simulink library "MFMbody_roadSurface"  (R2025a)
settings: Solver=VariableStepAuto  StartTime=0.0  StopTime=10.0  RelTol=1e-3
undefined symbols (not defined in the file): fcontactpatch, LorR, road_file, Scene, SceneData, Vehicle, X, Y, Z
libraries: sm_lib x21, nesl_utility x12, $bdroot x7
Description:
  | Component of Simscape Vehicle Templates Library
  | 
  | Copyright 2018-2026 The MathWorks, Inc.
settings Model: Creator=smiller  LastModifiedBy=smiller
settings OptimizationCC: ReuseModelBlockBuffer=off
settings ModelReferenceCC: EnableRefExpFcnMdlSchedulingChecks=on
settings RTWCC: GPUComputeCapability=3.5

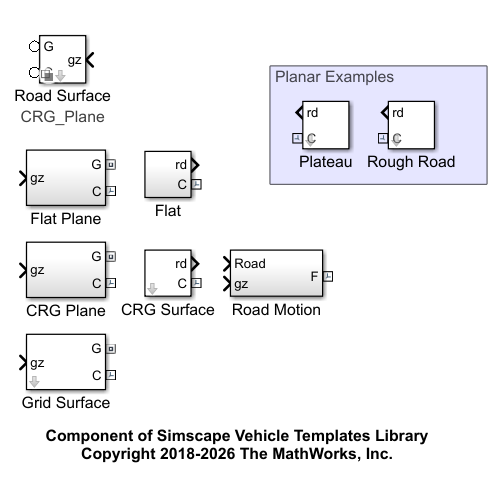
[thumbnail: Simulink's stored preview of the top-level diagram]
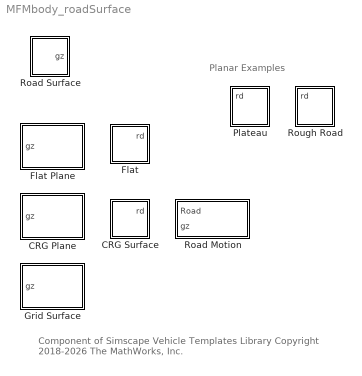
== system MFMbody_roadSurface ==
  note: Planar Examples
  note: Component of Simscape Vehicle Templates Library
      | Copyright 2018-2026 The MathWorks, Inc.
  CRG Plane : Subsystem
  CRG Surface : Subsystem  mask{road_file=road_file, LRind=LorR}
      mask prompts: road_file "Road File Name"; LRind "Index for Left (1) or Right (2)"
      mask init:
      | set_param([gcb '/Contact Plane'],'crg_file',road_file);
  Flat : Subsystem
  Flat Plane : Subsystem
  Grid Surface : Subsystem  mask{grid_file=Vehicle.Chassis.TireA1.roadFile.Value}
      mask prompts: grid_file "Road File Name (stl)"
      mask init:
      | parStr = ['Scene.' strrep(grid_file,'.stl','.gsd')];
      | 
      | set_param([gcb '/Grid Surface'],...
      |     'XGridVector',[parStr '.xg'],...
      |     'YGridVector',[parStr '.yg'],...
      |     'ZHeights',[parStr '.z_heights']);
  Plateau : Subsystem  mask{LRind=LorR}
      mask prompts: LRind "Index for Left (1) or Right (2)"
  Road Motion : Subsystem
  Road Surface : Subsystem  Variant=on  VariantControlMode=label  VariantControl=Choice  LabelModeActiveChoice=CRG_Plane  mask{popup_leftRight=Left}
      mask prompts: popup_leftRight "Left/Right"
      mask init:
      | LorR = 1;
      | if(strcmpi(get_param(gcb,'popup_leftRight'),'right'))
      |     LorR = 2;
      | end
      settings: AttributesFormatString=%<LabelModeActiveChoice>
      mask TypeOptions popup_leftRight: Left | Right
      mask Display: disp(' ')
  Rough Road : Subsystem  mask{LRind=LorR}
      mask prompts: LRind "Index for Left (1) or Right (2)"

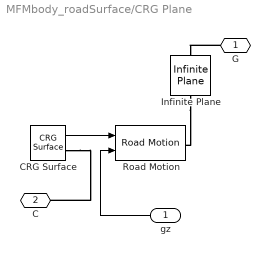
== system MFMbody_roadSurface/CRG Plane ==
  gz : Inport
  CRG Surface : $bdroot/CRG Surface  VariantControl=CRG_Surface  road_file=road_file  LRind=LorR
  Infinite Plane : sm_lib/Curves and Surfaces/Infinite Plane  GraphicType=Rectangle  GraphicPlaneWidth=1  GraphicPlaneWidthUnits=m  GraphicPlaneHeight=1  GraphicPlaneHeightUnits=m  GraphicVisPropType=SimpleVisualProperties  GraphicDiffuseColor=Visual.TireContactPlane.clr  GraphicOpacity=Visual.TireContactPlane.opc  GraphicSpecularColor=[0.5 0.5 0.5 1.0]  GraphicAmbientColor=[0.15 0.15 0.15 1.0]  GraphicEmissiveColor=[0.0 0.0 0.0 1.0]  GraphicShininess=75
  Road Motion : $bdroot/Road Motion  SystemSampleTime=-1  VariantActivationTime=update diagram  EmptyChoice=off  PassThrough=off  PassThroughVariantControl=(default)  EmptyChoiceVariantControl=(default)  AllowFlexibleInterface=on  Latency=0  AutoFrameSizeCalculation=off
  G : PMIOPort  Side=Right
  C : PMIOPort  Port=2  Side=Right
  wires:
  gz/1 -> Road Motion/2
  CRG Surface/1 -> Road Motion/1
  connections:
  CRG Surface/RConn1 -- C/RConn1
  Infinite Plane/LConn1 -- Road Motion/RConn1
  G/RConn1 -- Infinite Plane/RConn1

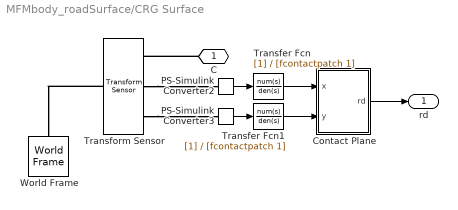
== system MFMbody_roadSurface/CRG Surface ==
  Contact Plane : Subsystem  mask{crg_file=road_file}
      mask prompts: crg_file "CRG Road File"
      mask init:
      | crg = crg_read(crg_file);
      | crg = rmfield(crg,'ct');
      | crg = rmfield(crg,'struct');
  PS-Simulink Converter2 : nesl_utility/PS-Simulink Converter  PhysicalDomain=network_engine_domain  SubClassName=ps_output  LeftPortType=input  RightPortType=output  PseudoPeriodic=off  Frequencies=[]  VectorFormat=inherit  Unit=inherit  AffineConversion=off
  PS-Simulink Converter3 : nesl_utility/PS-Simulink Converter  PhysicalDomain=network_engine_domain  SubClassName=ps_output  LeftPortType=input  RightPortType=output  PseudoPeriodic=off  Frequencies=[]  VectorFormat=inherit  Unit=inherit  AffineConversion=off
  Transfer Fcn : TransferFcn  Denominator=[fcontactpatch 1]
  Transfer Fcn1 : TransferFcn  Denominator=[fcontactpatch 1]
  Transform Sensor : sm_lib/Frames and Transforms/Transform Sensor  MeasurementFrame=World  RotationSequence=XYX  SenseAngle=off  SenseAxis=off  SenseQ=off  SenseR=off  SenseRotationSequence=off  SenseOmegaX=off  SenseOmegaY=off  SenseOmegaZ=off  SenseOmega=off  SenseQDot=off  SenseRDot=off  SenseRotationSequenceDot=off  SenseAlphaX=off  SenseAlphaY=off  SenseAlphaZ=off  SenseAlpha=off  SenseQDDot=off  SenseRDDot=off  SenseX=on  SenseY=on  SenseZ=off  SenseXYZ=off  SenseRad=off  SenseAzim=off  SenseDist=off  SenseInc=off  SenseXDot=off  SenseYDot=off  SenseZDot=off  SenseXYZDot=off  SenseRadDot=off  SenseAzimDot=off  SenseDistDot=off  SenseIncDot=off  SenseXDDot=off  SenseYDDot=off  SenseZDDot=off  SenseXYZDDot=off  SenseRadDDot=off  SenseAzimDDot=off  SenseDistDDot=off  SenseIncDDot=off
  World Frame : sm_lib/Frames and Transforms/World Frame
  C : PMIOPort  Side=Right
  rd : Outport
  wires:
  PS-Simulink Converter2/1 -> Transfer Fcn/1
  PS-Simulink Converter3/1 -> Transfer Fcn1/1
  Transfer Fcn/1 -> Contact Plane/1(x)
  Transfer Fcn1/1 -> Contact Plane/2(y)
  Contact Plane/1(rd) -> rd/1
  connections:
  Transform Sensor/LConn1 -- World Frame/RConn1
  Transform Sensor/RConn2 -- PS-Simulink Converter2/LConn1
  C/RConn1 -- Transform Sensor/RConn1
  Transform Sensor/RConn3 -- PS-Simulink Converter3/LConn1

== system MFMbody_roadSurface/Flat ==
  Reference Frame : sm_lib/Frames and Transforms/Reference Frame
  Road : Subsystem
  C : PMIOPort  Side=Right
  rd : Outport
  wires:
  Road/1(R) -> rd/1
  connections:
  C/RConn1 -- Reference Frame/RConn1

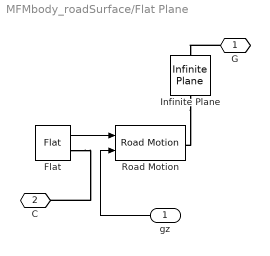
== system MFMbody_roadSurface/Flat Plane ==
  gz : Inport
  Flat : $bdroot/Flat  SystemSampleTime=-1  VariantControl=Flat  VariantActivationTime=update diagram  EmptyChoice=off  PassThrough=off  PassThroughVariantControl=(default)  EmptyChoiceVariantControl=(default)  AllowFlexibleInterface=on  Latency=0  AutoFrameSizeCalculation=off
  Infinite Plane : sm_lib/Curves and Surfaces/Infinite Plane  GraphicType=Rectangle  GraphicPlaneWidth=1  GraphicPlaneWidthUnits=m  GraphicPlaneHeight=1  GraphicPlaneHeightUnits=m  GraphicVisPropType=SimpleVisualProperties  GraphicDiffuseColor=Visual.TireContactPlane.clr  GraphicOpacity=Visual.TireContactPlane.opc  GraphicSpecularColor=[0.5 0.5 0.5 1.0]  GraphicAmbientColor=[0.15 0.15 0.15 1.0]  GraphicEmissiveColor=[0.0 0.0 0.0 1.0]  GraphicShininess=75
  Road Motion : $bdroot/Road Motion  SystemSampleTime=-1  VariantActivationTime=update diagram  EmptyChoice=off  PassThrough=off  PassThroughVariantControl=(default)  EmptyChoiceVariantControl=(default)  AllowFlexibleInterface=on  Latency=0  AutoFrameSizeCalculation=off
  G : PMIOPort  Side=Right
  C : PMIOPort  Port=2  Side=Right
  wires:
  Flat/1 -> Road Motion/1
  gz/1 -> Road Motion/2
  connections:
  G/RConn1 -- Infinite Plane/RConn1
  Infinite Plane/LConn1 -- Road Motion/RConn1
  Flat/RConn1 -- C/RConn1

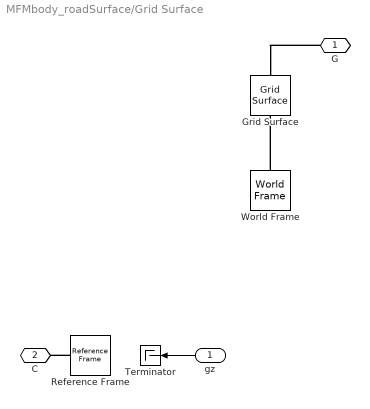
== system MFMbody_roadSurface/Grid Surface ==
  gz : Inport
  Grid Surface : sm_lib/Curves and Surfaces/Grid Surface  XGridVector=Scene.which('TNO_FlatRoad.rdf').xg  XGridVectorUnits=m  YGridVector=Scene.which('TNO_FlatRoad.rdf').yg  YGridVectorUnits=m  ZHeights=Scene.which('TNO_FlatRoad.rdf').z_heights  ZHeightsUnits=m  GraphicType=None  GraphicVisPropType=SimpleVisualProperties  GraphicDiffuseColor=[0.5 0.5 0.5]  GraphicOpacity=1  GraphicSpecularColor=[0.5 0.5 0.5 1.0]  GraphicAmbientColor=[0.15 0.15 0.15 1.0]  GraphicEmissiveColor=[0.0 0.0 0.0 1.0]  GraphicShininess=75
  Reference Frame : sm_lib/Frames and Transforms/Reference Frame
  Terminator : Terminator
  World Frame : sm_lib/Frames and Transforms/World Frame
  G : PMIOPort  Side=Right
  C : PMIOPort  Port=2  Side=Right
  wires:
  gz/1 -> Terminator/1
  connections:
  G/RConn1 -- Grid Surface/RConn1
  Reference Frame/RConn1 -- C/RConn1
  World Frame/RConn1 -- Grid Surface/LConn1

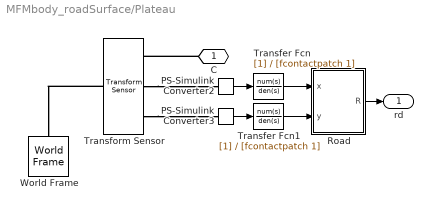
== system MFMbody_roadSurface/Plateau ==
  PS-Simulink Converter2 : nesl_utility/PS-Simulink Converter  PhysicalDomain=network_engine_domain  SubClassName=ps_output  LeftPortType=input  RightPortType=output  PseudoPeriodic=off  Frequencies=[]  VectorFormat=inherit  Unit=inherit  AffineConversion=off
  PS-Simulink Converter3 : nesl_utility/PS-Simulink Converter  PhysicalDomain=network_engine_domain  SubClassName=ps_output  LeftPortType=input  RightPortType=output  PseudoPeriodic=off  Frequencies=[]  VectorFormat=inherit  Unit=inherit  AffineConversion=off
  Road : Subsystem
  Transfer Fcn : TransferFcn  Denominator=[fcontactpatch 1]
  Transfer Fcn1 : TransferFcn  Denominator=[fcontactpatch 1]
  Transform Sensor : sm_lib/Frames and Transforms/Transform Sensor  MeasurementFrame=World  RotationSequence=XYX  SenseAngle=off  SenseAxis=off  SenseQ=off  SenseR=off  SenseRotationSequence=off  SenseOmegaX=off  SenseOmegaY=off  SenseOmegaZ=off  SenseOmega=off  SenseQDot=off  SenseRDot=off  SenseRotationSequenceDot=off  SenseAlphaX=off  SenseAlphaY=off  SenseAlphaZ=off  SenseAlpha=off  SenseQDDot=off  SenseRDDot=off  SenseX=on  SenseY=on  SenseZ=off  SenseXYZ=off  SenseRad=off  SenseAzim=off  SenseDist=off  SenseInc=off  SenseXDot=off  SenseYDot=off  SenseZDot=off  SenseXYZDot=off  SenseRadDot=off  SenseAzimDot=off  SenseDistDot=off  SenseIncDot=off  SenseXDDot=off  SenseYDDot=off  SenseZDDot=off  SenseXYZDDot=off  SenseRadDDot=off  SenseAzimDDot=off  SenseDistDDot=off  SenseIncDDot=off
  World Frame : sm_lib/Frames and Transforms/World Frame
  C : PMIOPort  Side=Right
  rd : Outport
  wires:
  PS-Simulink Converter2/1 -> Transfer Fcn/1
  PS-Simulink Converter3/1 -> Transfer Fcn1/1
  Road/1(R) -> rd/1
  Transfer Fcn/1 -> Road/1(x)
  Transfer Fcn1/1 -> Road/2(y)
  connections:
  Transform Sensor/LConn1 -- World Frame/RConn1
  Transform Sensor/RConn2 -- PS-Simulink Converter2/LConn1
  C/RConn1 -- Transform Sensor/RConn1
  Transform Sensor/RConn3 -- PS-Simulink Converter3/LConn1

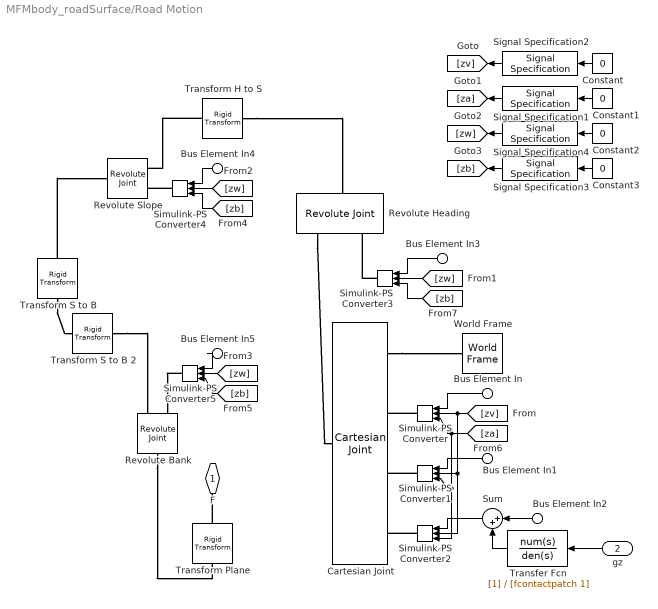
== system MFMbody_roadSurface/Road Motion ==
  Bus Element In : Inport  PortName=Road  Element=px
  Bus Element In1 : Inport  PortName=Road  Element=py
  Bus Element In2 : Inport  PortName=Road  Element=pz
  Bus Element In3 : Inport  PortName=Road  Element=qz
  Bus Element In4 : Inport  PortName=Road  Element=qy
  Bus Element In5 : Inport  PortName=Road  Element=qx
  gz : Inport  Port=2
  Cartesian Joint : sm_lib/Joints/Cartesian Joint  JointMode=Normal  CompositeWrenchDir=FollowerOnBase  CompositeWrenchFrame=BaseFrame  SenseConstraintForce=off  SenseConstraintTorque=off  SenseTotalForce=off  SenseTotalTorque=off  PxPositionTargetSpecify=off  PxPositionTargetPriority=High  PxPositionTargetValue=0  PxPositionTargetValueUnits=m  PxVelocityTargetSpecify=off  PxVelocityTargetPriority=High  PxVelocityTargetValue=0  PxVelocityTargetValueUnits=m/s  PxEquilibriumPosition=0  PxEquilibriumPositionUnits=m  PxSpringStiffness=0  PxSpringStiffnessUnits=N/m  PxDampingCoefficient=0  PxDampingCoefficientUnits=N/(m/s)  PxLowerLimitSpecify=off  PxLowerLimitBound=-1  PxLowerLimitBoundUnits=m  PxLowerLimitStiffness=1e6  PxLowerLimitStiffnessUnits=N/m  PxLowerLimitDamping=1e3  PxLowerLimitDampingUnits=N/(m/s)  PxLowerLimitTransitionRegionWidth=1e-4  PxLowerLimitTransitionRegionWidthUnits=m  PxUpperLimitSpecify=off  PxUpperLimitBound=1  PxUpperLimitBoundUnits=m  PxUpperLimitStiffness=1e6  PxUpperLimitStiffnessUnits=N/m  PxUpperLimitDamping=1e3  PxUpperLimitDampingUnits=N/(m/s)  PxUpperLimitTransitionRegionWidth=1e-4  PxUpperLimitTransitionRegionWidthUnits=m  PxTorqueActuationMode=ComputedTorque  PxMotionActuationMode=InputMotion  PxSensePosition=off  PxSenseVelocity=off  PxSenseAcceleration=off  PxSenseTorqueForce=off  PxSenseLowerLimitTorqueForce=off  PxSenseUpperLimitTorqueForce=off  PyPositionTargetSpecify=off  PyPositionTargetPriority=High  PyPositionTargetValue=0  PyPositionTargetValueUnits=m  PyVelocityTargetSpecify=off  PyVelocityTargetPriority=High  PyVelocityTargetValue=0  PyVelocityTargetValueUnits=m/s  PyEquilibriumPosition=0  PyEquilibriumPositionUnits=m  PySpringStiffness=0  PySpringStiffnessUnits=N/m  PyDampingCoefficient=0  PyDampingCoefficientUnits=N/(m/s)  PyLowerLimitSpecify=off  PyLowerLimitBound=-1  PyLowerLimitBoundUnits=m  PyLowerLimitStiffness=1e6  PyLowerLimitStiffnessUnits=N/m  PyLowerLimitDamping=1e3  PyLowerLimitDampingUnits=N/(m/s)  PyLowerLimitTransitionRegionWidth=1e-4  PyLowerLimitTransitionRegionWidthUnits=m  PyUpperLimitSpecify=off  PyUpperLimitBound=1  PyUpperLimitBoundUnits=m  PyUpperLimitStiffness=1e6  PyUpperLimitStiffnessUnits=N/m  PyUpperLimitDamping=1e3  PyUpperLimitDampingUnits=N/(m/s)  PyUpperLimitTransitionRegionWidth=1e-4  PyUpperLimitTransitionRegionWidthUnits=m  PyTorqueActuationMode=ComputedTorque  PyMotionActuationMode=InputMotion  PySensePosition=off  PySenseVelocity=off  PySenseAcceleration=off  PySenseTorqueForce=off  PySenseLowerLimitTorqueForce=off  PySenseUpperLimitTorqueForce=off  PzPositionTargetSpecify=off  PzPositionTargetPriority=High  PzPositionTargetValue=0  PzPositionTargetValueUnits=m  PzVelocityTargetSpecify=off  PzVelocityTargetPriority=High  PzVelocityTargetValue=0  PzVelocityTargetValueUnits=m/s  PzEquilibriumPosition=0  PzEquilibriumPositionUnits=m  PzSpringStiffness=0  PzSpringStiffnessUnits=N/m  PzDampingCoefficient=0  PzDampingCoefficientUnits=N/(m/s)  PzLowerLimitSpecify=off  PzLowerLimitBound=-1  PzLowerLimitBoundUnits=m  PzLowerLimitStiffness=1e6  PzLowerLimitStiffnessUnits=N/m  PzLowerLimitDamping=1e3  PzLowerLimitDampingUnits=N/(m/s)  PzLowerLimitTransitionRegionWidth=1e-4  PzLowerLimitTransitionRegionWidthUnits=m  PzUpperLimitSpecify=off  PzUpperLimitBound=1  PzUpperLimitBoundUnits=m  PzUpperLimitStiffness=1e6  PzUpperLimitStiffnessUnits=N/m  PzUpperLimitDamping=1e3  PzUpperLimitDampingUnits=N/(m/s)  PzUpperLimitTransitionRegionWidth=1e-4  PzUpperLimitTransitionRegionWidthUnits=m  PzTorqueActuationMode=ComputedTorque  PzMotionActuationMode=InputMotion  PzSensePosition=off  PzSenseVelocity=off  PzSenseAcceleration=off  PzSenseTorqueForce=off  PzSenseLowerLimitTorqueForce=off  PzSenseUpperLimitTorqueForce=off
  Constant{,1..3} (4 alike) : Constant  Value=0
  Revolute Heading : sm_lib/Joints/Revolute Joint  JointMode=Normal  CompositeWrenchDir=FollowerOnBase  CompositeWrenchFrame=BaseFrame  SenseConstraintForce=off  SenseConstraintTorque=off  SenseTotalForce=off  SenseTotalTorque=off  PositionTargetSpecify=off  PositionTargetPriority=High  PositionTargetValue=0  PositionTargetValueUnits=deg  VelocityTargetSpecify=off  VelocityTargetPriority=High  VelocityTargetValue=0  VelocityTargetValueUnits=deg/s  EquilibriumPosition=0  EquilibriumPositionUnits=deg  SpringStiffness=0  SpringStiffnessUnits=N*m/deg  DampingCoefficient=0  DampingCoefficientUnits=N*m/(deg/s)  LowerLimitSpecify=off  LowerLimitBound=-90  LowerLimitBoundUnits=deg  LowerLimitStiffness=1e4  LowerLimitStiffnessUnits=N*m/deg  LowerLimitDamping=10  LowerLimitDampingUnits=N*m/(deg/s)  LowerLimitTransitionRegionWidth=0.1  LowerLimitTransitionRegionWidthUnits=deg  UpperLimitSpecify=off  UpperLimitBound=90  UpperLimitBoundUnits=deg  UpperLimitStiffness=1e4  UpperLimitStiffnessUnits=N*m/deg  UpperLimitDamping=10  UpperLimitDampingUnits=N*m/(deg/s)  UpperLimitTransitionRegionWidth=0.1  UpperLimitTransitionRegionWidthUnits=deg  TorqueActuationMode=ComputedTorque  MotionActuationMode=InputMotion  SensePosition=off  SenseVelocity=off  SenseAcceleration=off  SenseTorqueForce=off  SenseLowerLimitTorqueForce=off  SenseUpperLimitTorqueForce=off
  Revolute Slope : sm_lib/Joints/Revolute Joint  JointMode=Normal  CompositeWrenchDir=FollowerOnBase  CompositeWrenchFrame=BaseFrame  SenseConstraintForce=off  SenseConstraintTorque=off  SenseTotalForce=off  SenseTotalTorque=off  PositionTargetSpecify=off  PositionTargetPriority=High  PositionTargetValue=0  PositionTargetValueUnits=deg  VelocityTargetSpecify=off  VelocityTargetPriority=High  VelocityTargetValue=0  VelocityTargetValueUnits=deg/s  EquilibriumPosition=0  EquilibriumPositionUnits=deg  SpringStiffness=0  SpringStiffnessUnits=N*m/deg  DampingCoefficient=0  DampingCoefficientUnits=N*m/(deg/s)  LowerLimitSpecify=off  LowerLimitBound=-90  LowerLimitBoundUnits=deg  LowerLimitStiffness=1e4  LowerLimitStiffnessUnits=N*m/deg  LowerLimitDamping=10  LowerLimitDampingUnits=N*m/(deg/s)  LowerLimitTransitionRegionWidth=0.1  LowerLimitTransitionRegionWidthUnits=deg  UpperLimitSpecify=off  UpperLimitBound=90  UpperLimitBoundUnits=deg  UpperLimitStiffness=1e4  UpperLimitStiffnessUnits=N*m/deg  UpperLimitDamping=10  UpperLimitDampingUnits=N*m/(deg/s)  UpperLimitTransitionRegionWidth=0.1  UpperLimitTransitionRegionWidthUnits=deg  TorqueActuationMode=ComputedTorque  MotionActuationMode=InputMotion  SensePosition=off  SenseVelocity=off  SenseAcceleration=off  SenseTorqueForce=off  SenseLowerLimitTorqueForce=off  SenseUpperLimitTorqueForce=off
  Revolute Bank : sm_lib/Joints/Revolute Joint  JointMode=Normal  CompositeWrenchDir=FollowerOnBase  CompositeWrenchFrame=BaseFrame  SenseConstraintForce=off  SenseConstraintTorque=off  SenseTotalForce=off  SenseTotalTorque=off  PositionTargetSpecify=off  PositionTargetPriority=High  PositionTargetValue=0  PositionTargetValueUnits=deg  VelocityTargetSpecify=off  VelocityTargetPriority=High  VelocityTargetValue=0  VelocityTargetValueUnits=deg/s  EquilibriumPosition=0  EquilibriumPositionUnits=deg  SpringStiffness=0  SpringStiffnessUnits=N*m/deg  DampingCoefficient=0  DampingCoefficientUnits=N*m/(deg/s)  LowerLimitSpecify=off  LowerLimitBound=-90  LowerLimitBoundUnits=deg  LowerLimitStiffness=1e4  LowerLimitStiffnessUnits=N*m/deg  LowerLimitDamping=10  LowerLimitDampingUnits=N*m/(deg/s)  LowerLimitTransitionRegionWidth=0.1  LowerLimitTransitionRegionWidthUnits=deg  UpperLimitSpecify=off  UpperLimitBound=90  UpperLimitBoundUnits=deg  UpperLimitStiffness=1e4  UpperLimitStiffnessUnits=N*m/deg  UpperLimitDamping=10  UpperLimitDampingUnits=N*m/(deg/s)  UpperLimitTransitionRegionWidth=0.1  UpperLimitTransitionRegionWidthUnits=deg  TorqueActuationMode=ComputedTorque  MotionActuationMode=InputMotion  SensePosition=off  SenseVelocity=off  SenseAcceleration=off  SenseTorqueForce=off  SenseLowerLimitTorqueForce=off  SenseUpperLimitTorqueForce=off
  Signal Specification1 : SignalSpecification  Unit=m/s^2
  Signal Specification2 : SignalSpecification  Unit=m/s
  Signal Specification3 : SignalSpecification  Unit=rad/s^2
  Signal Specification4 : SignalSpecification  Unit=rad/s
  Simulink-PS Converter : nesl_utility/Simulink-PS Converter  PhysicalDomain=network_engine_domain  SubClassName=ps_input  LeftPortType=input  RightPortType=output  PseudoPeriodic=off  Frequencies=[]  NoiseDistribution=none  NoiseParameters=[]  Unit=m  AffineConversion=off  FilteringAndDerivatives=provide  SimscapeFilterOrder=1  InputFilterTimeConstant=0.001  UdotUserProvided=2
  Simulink-PS Converter1 : nesl_utility/Simulink-PS Converter  PhysicalDomain=network_engine_domain  SubClassName=ps_input  LeftPortType=input  RightPortType=output  PseudoPeriodic=off  Frequencies=[]  NoiseDistribution=none  NoiseParameters=[]  Unit=m  AffineConversion=off  FilteringAndDerivatives=provide  SimscapeFilterOrder=1  InputFilterTimeConstant=0.001  UdotUserProvided=2
  Simulink-PS Converter2 : nesl_utility/Simulink-PS Converter  PhysicalDomain=network_engine_domain  SubClassName=ps_input  LeftPortType=input  RightPortType=output  PseudoPeriodic=off  Frequencies=[]  NoiseDistribution=none  NoiseParameters=[]  Unit=m  AffineConversion=off  FilteringAndDerivatives=provide  SimscapeFilterOrder=1  InputFilterTimeConstant=0.001  UdotUserProvided=2
  Simulink-PS Converter3 : nesl_utility/Simulink-PS Converter  PhysicalDomain=network_engine_domain  SubClassName=ps_input  LeftPortType=input  RightPortType=output  PseudoPeriodic=off  Frequencies=[]  NoiseDistribution=none  NoiseParameters=[]  Unit=rad  AffineConversion=off  FilteringAndDerivatives=provide  SimscapeFilterOrder=1  InputFilterTimeConstant=0.001  UdotUserProvided=2
  Simulink-PS Converter4 : nesl_utility/Simulink-PS Converter  PhysicalDomain=network_engine_domain  SubClassName=ps_input  LeftPortType=input  RightPortType=output  PseudoPeriodic=off  Frequencies=[]  NoiseDistribution=none  NoiseParameters=[]  Unit=rad  AffineConversion=off  FilteringAndDerivatives=provide  SimscapeFilterOrder=1  InputFilterTimeConstant=0.001  UdotUserProvided=2
  Simulink-PS Converter5 : nesl_utility/Simulink-PS Converter  PhysicalDomain=network_engine_domain  SubClassName=ps_input  LeftPortType=input  RightPortType=output  PseudoPeriodic=off  Frequencies=[]  NoiseDistribution=none  NoiseParameters=[]  Unit=rad  AffineConversion=off  FilteringAndDerivatives=provide  SimscapeFilterOrder=1  InputFilterTimeConstant=0.001  UdotUserProvided=2
  Sum : Sum  Inputs=|++
  Transfer Fcn : TransferFcn  Denominator=[fcontactpatch 1]
  Transform H to S : sm_lib/Frames and Transforms/Rigid Transform  RotationMethod=AlignedAxes  FollAlignAxisA=+Z  BaseAlignAxisA=+Y  FollAlignAxisB=+X  BaseAlignAxisB=+X  RotationStandardAxis=+Z  RotationAngle=0.0  RotationAngleUnits=deg  RotationArbitraryAxis=[0 0 1]  RotationSequenceAxes=FollowerAxes  RotationSequence=XYX  RotationSequenceAngles=[0 0 0]  RotationSequenceAnglesUnits=deg  RotationMatrix=[1 0 0; 0 1 0; 0 0 1]  Quaternion=[1 0 0 0]  TranslationMethod=None  TranslationCartesianOffset=[0 0 0]  TranslationCartesianOffsetUnits=m  TranslationStandardAxis=+Z  TranslationStandardOffset=0  TranslationStandardOffsetUnits=m  TranslationROffset=0  TranslationROffsetUnits=m  TranslationThetaOffset=0  TranslationThetaOffsetUnits=deg  TranslationZOffset=0  TranslationZOffsetUnits=m
  Transform Plane : sm_lib/Frames and Transforms/Rigid Transform  RotationMethod=AlignedAxes  FollAlignAxisA=+Z  BaseAlignAxisA=-X  FollAlignAxisB=+Y  BaseAlignAxisB=+Y  RotationStandardAxis=+Z  RotationAngle=0.0  RotationAngleUnits=deg  RotationArbitraryAxis=[0 0 1]  RotationSequenceAxes=FollowerAxes  RotationSequence=XYX  RotationSequenceAngles=[0 0 0]  RotationSequenceAnglesUnits=deg  RotationMatrix=[1 0 0; 0 1 0; 0 0 1]  Quaternion=[1 0 0 0]  TranslationMethod=None  TranslationCartesianOffset=[0 0 0]  TranslationCartesianOffsetUnits=m  TranslationStandardAxis=+Z  TranslationStandardOffset=0  TranslationStandardOffsetUnits=m  TranslationROffset=0  TranslationROffsetUnits=m  TranslationThetaOffset=0  TranslationThetaOffsetUnits=deg  TranslationZOffset=0  TranslationZOffsetUnits=m
  Transform S to B : sm_lib/Frames and Transforms/Rigid Transform  RotationMethod=AlignedAxes  FollAlignAxisA=+Z  BaseAlignAxisA=-Y  FollAlignAxisB=+X  BaseAlignAxisB=+X  RotationStandardAxis=+Z  RotationAngle=0.0  RotationAngleUnits=deg  RotationArbitraryAxis=[0 0 1]  RotationSequenceAxes=FollowerAxes  RotationSequence=XYX  RotationSequenceAngles=[0 0 0]  RotationSequenceAnglesUnits=deg  RotationMatrix=[1 0 0; 0 1 0; 0 0 1]  Quaternion=[1 0 0 0]  TranslationMethod=None  TranslationCartesianOffset=[0 0 0]  TranslationCartesianOffsetUnits=m  TranslationStandardAxis=+Z  TranslationStandardOffset=0  TranslationStandardOffsetUnits=m  TranslationROffset=0  TranslationROffsetUnits=m  TranslationThetaOffset=0  TranslationThetaOffsetUnits=deg  TranslationZOffset=0  TranslationZOffsetUnits=m
  Transform S to B 2 : sm_lib/Frames and Transforms/Rigid Transform  RotationMethod=AlignedAxes  FollAlignAxisA=+Z  BaseAlignAxisA=+X  FollAlignAxisB=+Y  BaseAlignAxisB=+Y  RotationStandardAxis=+Z  RotationAngle=0.0  RotationAngleUnits=deg  RotationArbitraryAxis=[0 0 1]  RotationSequenceAxes=FollowerAxes  RotationSequence=XYX  RotationSequenceAngles=[0 0 0]  RotationSequenceAnglesUnits=deg  RotationMatrix=[1 0 0; 0 1 0; 0 0 1]  Quaternion=[1 0 0 0]  TranslationMethod=None  TranslationCartesianOffset=[0 0 0]  TranslationCartesianOffsetUnits=m  TranslationStandardAxis=+Z  TranslationStandardOffset=0  TranslationStandardOffsetUnits=m  TranslationROffset=0  TranslationROffsetUnits=m  TranslationThetaOffset=0  TranslationThetaOffsetUnits=deg  TranslationZOffset=0  TranslationZOffsetUnits=m
  World Frame : sm_lib/Frames and Transforms/World Frame
  F : PMIOPort  Side=Right
  wires:
  Constant2/1 -> Signal Specification4/1
  Constant3/1 -> Signal Specification3/1
  Signal Specification4/1 -> [zw]
  Signal Specification3/1 -> [zb]
  Signal Specification1/1 -> [za]
  Signal Specification2/1 -> [zv]
  [zb] -> Simulink-PS Converter3/3
  [za] -> Simulink-PS Converter1/3, Simulink-PS Converter2/3, Simulink-PS Converter/3
  [zb] -> Simulink-PS Converter5/3
  [zb] -> Simulink-PS Converter4/3
  Constant1/1 -> Signal Specification1/1
  [zw] -> Simulink-PS Converter3/2
  [zw] -> Simulink-PS Converter5/2
  [zv] -> Simulink-PS Converter1/2, Simulink-PS Converter2/2, Simulink-PS Converter/2
  [zw] -> Simulink-PS Converter4/2
  Constant/1 -> Signal Specification2/1
  Bus Element In5/1 -> Simulink-PS Converter5/1
  Bus Element In4/1 -> Simulink-PS Converter4/1
  Bus Element In3/1 -> Simulink-PS Converter3/1
  Sum/1 -> Simulink-PS Converter2/1
  Bus Element In1/1 -> Simulink-PS Converter1/1
  Bus Element In/1 -> Simulink-PS Converter/1
  Bus Element In2/1 -> Sum/1
  gz/1 -> Transfer Fcn/1
  Transfer Fcn/1 -> Sum/2
  connections:
  Simulink-PS Converter2/RConn1 -- Cartesian Joint/LConn4
  Simulink-PS Converter5/RConn1 -- Revolute Bank/LConn2
  Simulink-PS Converter3/RConn1 -- Revolute Heading/LConn2
  Cartesian Joint/LConn1 -- World Frame/RConn1
  Simulink-PS Converter4/RConn1 -- Revolute Slope/LConn2
  Simulink-PS Converter/RConn1 -- Cartesian Joint/LConn2
  Transform S to B/RConn1 -- Transform S to B 2/LConn1
  Transform S to B 2/RConn1 -- Revolute Bank/LConn1
  Transform S to B/LConn1 -- Revolute Slope/RConn1
  Revolute Heading/LConn1 -- Cartesian Joint/RConn1
  Simulink-PS Converter1/RConn1 -- Cartesian Joint/LConn3
  Transform Plane/RConn1 -- F/RConn1
  Revolute Bank/RConn1 -- Transform Plane/LConn1
  Transform H to S/LConn1 -- Revolute Heading/RConn1
  Transform H to S/RConn1 -- Revolute Slope/LConn1

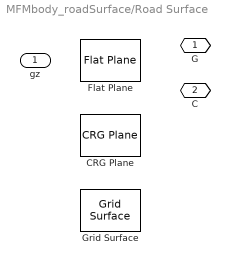
== system MFMbody_roadSurface/Road Surface ==
  gz : Inport
  CRG Plane : $bdroot/CRG Plane  SystemSampleTime=-1  VariantControl=CRG_Plane  VariantActivationTime=update diagram  EmptyChoice=off  PassThrough=off  PassThroughVariantControl=(default)  EmptyChoiceVariantControl=(default)  AllowFlexibleInterface=on  Latency=0  AutoFrameSizeCalculation=off
  Flat Plane : $bdroot/Flat Plane  SystemSampleTime=-1  VariantControl=Flat_Plane  VariantActivationTime=update diagram  EmptyChoice=off  PassThrough=off  PassThroughVariantControl=(default)  EmptyChoiceVariantControl=(default)  AllowFlexibleInterface=on  Latency=0  AutoFrameSizeCalculation=off
  Grid Surface : $bdroot/Grid Surface  VariantControl=Grid_Surface  grid_file=road_file
  G : PMIOPort  Side=Right
  C : PMIOPort  Port=2  Side=Right

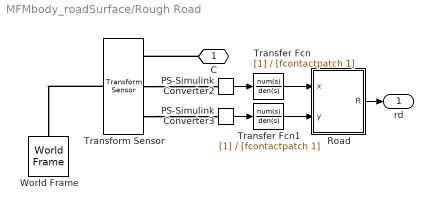
== system MFMbody_roadSurface/Rough Road ==
  PS-Simulink Converter2 : nesl_utility/PS-Simulink Converter  PhysicalDomain=network_engine_domain  SubClassName=ps_output  LeftPortType=input  RightPortType=output  PseudoPeriodic=off  Frequencies=[]  VectorFormat=inherit  Unit=inherit  AffineConversion=off
  PS-Simulink Converter3 : nesl_utility/PS-Simulink Converter  PhysicalDomain=network_engine_domain  SubClassName=ps_output  LeftPortType=input  RightPortType=output  PseudoPeriodic=off  Frequencies=[]  VectorFormat=inherit  Unit=inherit  AffineConversion=off
  Road : Subsystem
  Transfer Fcn : TransferFcn  Denominator=[fcontactpatch 1]
  Transfer Fcn1 : TransferFcn  Denominator=[fcontactpatch 1]
  Transform Sensor : sm_lib/Frames and Transforms/Transform Sensor  MeasurementFrame=World  RotationSequence=XYX  SenseAngle=off  SenseAxis=off  SenseQ=off  SenseR=off  SenseRotationSequence=off  SenseOmegaX=off  SenseOmegaY=off  SenseOmegaZ=off  SenseOmega=off  SenseQDot=off  SenseRDot=off  SenseRotationSequenceDot=off  SenseAlphaX=off  SenseAlphaY=off  SenseAlphaZ=off  SenseAlpha=off  SenseQDDot=off  SenseRDDot=off  SenseX=on  SenseY=on  SenseZ=off  SenseXYZ=off  SenseRad=off  SenseAzim=off  SenseDist=off  SenseInc=off  SenseXDot=off  SenseYDot=off  SenseZDot=off  SenseXYZDot=off  SenseRadDot=off  SenseAzimDot=off  SenseDistDot=off  SenseIncDot=off  SenseXDDot=off  SenseYDDot=off  SenseZDDot=off  SenseXYZDDot=off  SenseRadDDot=off  SenseAzimDDot=off  SenseDistDDot=off  SenseIncDDot=off
  World Frame : sm_lib/Frames and Transforms/World Frame
  C : PMIOPort  Side=Right
  rd : Outport
  wires:
  Transfer Fcn1/1 -> Road/2(y)
  Transfer Fcn/1 -> Road/1(x)
  Road/1(R) -> rd/1
  PS-Simulink Converter3/1 -> Transfer Fcn1/1
  PS-Simulink Converter2/1 -> Transfer Fcn/1
  connections:
  Transform Sensor/RConn3 -- PS-Simulink Converter3/LConn1
  C/RConn1 -- Transform Sensor/RConn1
  Transform Sensor/RConn2 -- PS-Simulink Converter2/LConn1
  Transform Sensor/LConn1 -- World Frame/RConn1

== system MFMbody_roadSurface/CRG Surface/Contact Plane ==
  x : Inport
  y : Inport  Port=2
  Bus Creator1 : BusCreator  Inputs=6
  CRG to Contact Plane : MATLAB Function  TreatAsAtomicUnit=on
  rd : Outport
  wires:
  y/1 -> CRG to Contact Plane/2(y)
  x/1 -> CRG to Contact Plane/1(x)
  Bus Creator1/1 -> rd/1
  CRG to Contact Plane/1(px) -> Bus Creator1/1  "px"
  CRG to Contact Plane/2(py) -> Bus Creator1/2  "py"
  CRG to Contact Plane/3(pz) -> Bus Creator1/3  "pz"
  CRG to Contact Plane/4(qx) -> Bus Creator1/4  "qx"
  CRG to Contact Plane/5(qy) -> Bus Creator1/5  "qy"
  CRG to Contact Plane/6(qz) -> Bus Creator1/6  "qz"

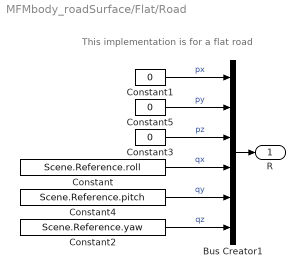
== system MFMbody_roadSurface/Flat/Road ==
  note: This implementation is for a flat road
  Bus Creator1 : BusCreator  Inputs=6
  Constant : Constant  Value=Scene.Reference.roll
  Constant1 : Constant  Value=0
  Constant2 : Constant  Value=Scene.Reference.yaw
  Constant3 : Constant  Value=0
  Constant4 : Constant  Value=Scene.Reference.pitch
  Constant5 : Constant  Value=0
  R : Outport
  wires:
  Constant4/1 -> Bus Creator1/5  "qy"
  Bus Creator1/1 -> R/1
  Constant2/1 -> Bus Creator1/6  "qz"
  Constant/1 -> Bus Creator1/4  "qx"
  Constant5/1 -> Bus Creator1/2  "py"
  Constant3/1 -> Bus Creator1/3  "pz"
  Constant1/1 -> Bus Creator1/1  "px"

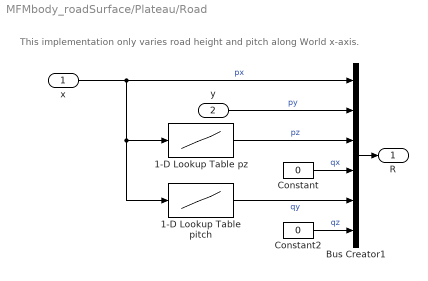
== system MFMbody_roadSurface/Plateau/Road ==
  note: This implementation only varies road height and pitch along World x-axis.
  x : Inport
  y : Inport  Port=2
  1-D Lookup Table pitch : Lookup_n-D  NumberOfTableDimensions=1  BreakpointsForDimension1=SceneData.Plateau.Road.qyLUT.px  Table=SceneData.Plateau.Road.qyLUT.qy(:,LRind)  InterpMethod=Akima spline  InternalRulePriority=Speed  RndMeth=Simplest
  1-D Lookup Table pz : Lookup_n-D  NumberOfTableDimensions=1  BreakpointsForDimension1=SceneData.Plateau.Road.pzLUT.px  Table=SceneData.Plateau.Road.pzLUT.pz(:,LRind)  InterpMethod=Akima spline  InternalRulePriority=Speed  RndMeth=Simplest
  Bus Creator1 : BusCreator  Inputs=6
  Constant : Constant  Value=0
  Constant2 : Constant  Value=0
  R : Outport
  wires:
  x/1 -> Bus Creator1/1, 1-D Lookup Table pz/1, 1-D Lookup Table pitch/1  "px"
  y/1 -> Bus Creator1/2  "py"
  Constant/1 -> Bus Creator1/4  "qx"
  Constant2/1 -> Bus Creator1/6  "qz"
  Bus Creator1/1 -> R/1
  1-D Lookup Table pitch/1 -> Bus Creator1/5  "qy"
  1-D Lookup Table pz/1 -> Bus Creator1/3  "pz"

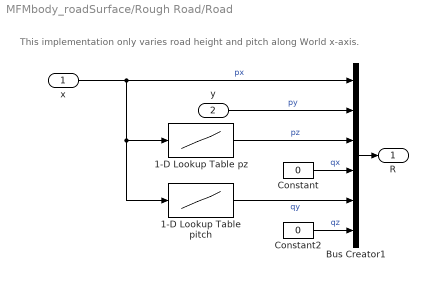
== system MFMbody_roadSurface/Rough Road/Road ==
  note: This implementation only varies road height and pitch along World x-axis.
  x : Inport
  y : Inport  Port=2
  1-D Lookup Table pitch : Lookup_n-D  NumberOfTableDimensions=1  BreakpointsForDimension1=SceneData.Rough_Road.Road.qyLUT.px  Table=SceneData.Rough_Road.Road.qyLUT.qy(:,LRind)  InterpMethod=Akima spline  InternalRulePriority=Speed  RndMeth=Simplest
  1-D Lookup Table pz : Lookup_n-D  NumberOfTableDimensions=1  BreakpointsForDimension1=SceneData.Rough_Road.Road.pzLUT.px  Table=SceneData.Rough_Road.Road.pzLUT.pz(:,LRind)  InterpMethod=Akima spline  InternalRulePriority=Speed  RndMeth=Simplest
  Bus Creator1 : BusCreator  Inputs=6
  Constant : Constant  Value=0
  Constant2 : Constant  Value=0
  R : Outport
  wires:
  1-D Lookup Table pz/1 -> Bus Creator1/3  "pz"
  1-D Lookup Table pitch/1 -> Bus Creator1/5  "qy"
  Bus Creator1/1 -> R/1
  Constant2/1 -> Bus Creator1/6  "qz"
  Constant/1 -> Bus Creator1/4  "qx"
  y/1 -> Bus Creator1/2  "py"
  x/1 -> 1-D Lookup Table pitch/1, 1-D Lookup Table pz/1, Bus Creator1/1  "px"

== matlab function MFMbody_roadSurface/CRG Surface/Contact Plane/CRG to Contact Plane ==
  data: px output; py output; pz output; qx output; x input; y input; qy output; qz output; crg parameter
function [px, py, pz, qx, qy, qz] = fcn(x, y, crg)

% Assign default values for all quantities
px = x;
py = y;
pz = 0.0;
qx = 0.0;
qy = 0.0;
qz = 0.0;

% Use x-y position information to get
% u-v position in curved regular grid
pxy = [x, y];
[puv, crg] = crg_eval_xy2uv_codegen(crg, pxy);

%% Contact point height 
% Option one, obtain point
[pz, crg] = crg_eval_uv2z_codegen(crg, puv);

% Option two, get vector of points and interpolate
%puv_set = puv+[-5 0;-4 0;-3 0;-2 0;-0.5 0;0.5 0;1 0;2 0;3 0;4 0;5 0]*0.1;
%[pz_set, crg] = crg_eval_uv2z_codegen(crg, puv_set);
%crg_z = interp1(puv_set(:,1),pz_set,puv(1),'pchip');
%pz = double(crg_z);

%% Heading
% Option one - obtain curvature point
%[phi, crg] = crg_eval_u2phi(crg, puv(1));
%qz = phi;

% Option two - get set of points and interpolate
if(isfield(crg,'p'))
    crg_p = interp1([0:crg.head.uinc:crg.u],[crg.p(1) crg.p],puv(1),'pchip');
    qz = double(crg_p);
else
    qz=0;
end


%% Slope
% Option one - Obtain forward and backward height to estimate the slope
% 
%{
h = 1e-1;    % Distance forward/backward in m

xHigh = x + h * cos(qz);
yHigh = y + h * sin(qz);
[pzHigh, crg] = crg_eval_xy2z(crg, [xHigh, yHigh]);

xLow = x - h * cos(qz);
yLow = y - h * sin(qz);
[pzLow, ~] = crg_eval_xy2z(crg, [xLow, yLow]);

deriv = (pzHigh - pzLow) / sqrt(2 * h * h);
qy = -atan(deriv);
%}

% Option two, take average from a set
%{x
puv_set = puv+[-5 0;-4 0;-3 0;-2 0;-0.5 0;0.5 0;1 0;2 0;3 0;4 0;5 0]*0.1;
[pz_set, ~] = crg_eval_uv2z_codegen(crg, puv_set);
qy_set = atan(diff(pz_set)./diff(puv_set(:,1)));
qy = -mean(qy_set);
%

% Option three, interpolate from slope assigned in crg data set
%crg_s = interp1([0:crg.head.uinc:crg.u],[crg.s(1) crg.s],puv(1),'pchip');
%qy   = double(-atan(crg_s));
